simulink model "DCMotorOpenLoop"  (R2026b)
settings: Solver=FixedStepDiscrete  StopTime=OL_StopTime  FixedStep=Ts
PreLoadFcn:
  | DCMotorParams;
InitFcn:
  | DCMotorParams;
values from neighbouring files (symbols this model uses):
  OL_DutyGain = 1    [DCMotorParams.m]
libraries: simulink x1
settings Model: SILPILModeSetting=veronly  Creator=bence  LastModifiedBy=bence
settings SolverCC: AutoInsertRateTranBlk=on
settings OptimizationCC: DifferentSizesBufferReuse=on  EfficientTunableParamExpr=on  EnhancedBackFolding=on  MaxStackSize=64  OptimizationCustomize=off  OptimizeBlockOrder=speed  PassReuseOutputArgsAs=Individual arguments  RemoveInternalMemoryZeroInit=on  RemoveRootLevelIOMemoryZeroInit=on
settings DebuggingCC: ParameterTunabilityLossMsg=error
settings HardwareCC: ProdHWDeviceType=Atmel->AVR  ProdLargestAtomicFloat=None
settings SFSimCC: MATLABDynamicMemAlloc=off
settings RTWCC: BuildConfiguration=Faster Runs  Description=Embedded Coder  HardwareBoard=Arduino Uno  SystemTargetFile=ert.tlc  TLCOptions=-aInlineSetEventsForThisBaseRateFcn=TLC_FALSE -aSuppressMultiTaskScheduler=TLC_FALSE -aRateBasedStepFcn=1  TemplateMakefile=ert_default_tmf  Toolchain=Arduino AVR
settings CodeAppCC: ForceParamTrailComments=on  IgnoreCustomStorageClasses=off  InsertBlockDesc=on  OperatorAnnotations=on  SFDataObjDesc=on  SimulinkDataObjDesc=on
settings ERTTargetCC: CombineSignalStateStructs=on  ExtMode=on  ExtModeAutomaticAllocSize=off  ExtModeIntrfLevel=Level2 - Open  ExtModeMexFile=ext_xcp  ExtModeStaticAlloc=on  SupportContinuousTime=on  SupportVariableSizeSignals=on

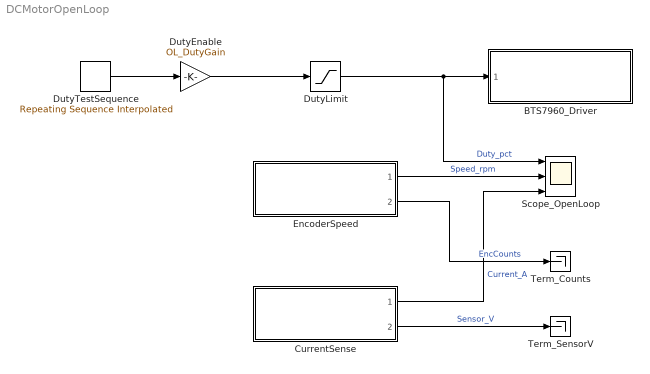
== system DCMotorOpenLoop ==
  BTS7960_Driver : Subsystem  ReferencedSubsystem=DC7960MDriver
  CurrentSense : Subsystem  ReferencedSubsystem=CurrentSense
  DutyEnable : Gain  Gain=OL_DutyGain
  DutyLimit : Saturate  UpperLimit=100  LowerLimit=-100
  DutyTestSequence : simulink/Sources/Repeating Sequence Interpolated  OutValues=OL_SeqDuty.'  TimeValues=OL_SeqTime.'  LookUpMeth=Use Input Below  tsamp=Ts  OutMin=[]  OutMax=[]  OutDataTypeStr=double  OutputDataTypeScalingMode=double  OutDataType=fixdt(0,8)  OutScaling=2^-10
  EncoderSpeed : Subsystem  ReferencedSubsystem=EncoderSpeed
  Scope_OpenLoop : Scope  NumInputPorts=3
      settings: ActiveDisplayYMinimum=1908.968699538437  ActiveDisplayYMaximum=2812.4083076941924
  Term_Counts : Terminator
  Term_SensorV : Terminator
  wires:
  CurrentSense/2 -> Term_SensorV/1  "Sensor_V"
  EncoderSpeed/2 -> Term_Counts/1  "EncCounts"
  CurrentSense/1 -> Scope_OpenLoop/3  "Current_A"
  EncoderSpeed/1 -> Scope_OpenLoop/2  "Speed_rpm"
  DutyLimit/1 -> BTS7960_Driver/1, Scope_OpenLoop/1  "Duty_pct"
  DutyEnable/1 -> DutyLimit/1
  DutyTestSequence/1 -> DutyEnable/1
